simulink model "jumeau_banc_rw"  (R2025b)
settings: Solver=ode23t  StartTime=0.0  StopTime=20  MaxStep=1e-3  RelTol=1e-4
PostLoadFcn:
  | d = fileparts(get_param('jumeau_banc_rw', 'FileName')); addpath(fullfile(d, 'geometrie'), fullfile(d, 'liaison'), fullfile(d, 'pilotage')); clear d
StartFcn:
  | % Jumeau Webots : au lancement, MATLAB envoie les paramètres du Model Workspace à Webots, qui remet le banc en
  | % position de départ, puis ouvre la liaison de télémétrie et la liaison de commande (liaison/pont_banc.m).
  | if strcmp(get_param('jumeau_banc_rw/Procédé', 'LabelModeActiveChoice'), 'Webots')
  |     pont_banc('ouvrir', getVariable(get_param('jumeau_banc_rw', 'ModelWorkspace'), 'config_jumeau'));
  | end
  | pilotage_banc('depart');   % interface de pilotage : nouveau lancement
StopFcn:
  | pont_banc('fermer');
  | pilotage_banc('fin');
model workspace (MATLAB code in the model file):
  | %% Jumeau numérique du banc de stabilisation à 4 roues de réaction (version 3) : paramètres
  | % Ce code est enregistré dans le modèle (Model Explorer > jumeau_banc_rw > Model Workspace).
  | % Origine : (CAO) CAO du banc version 3, (M) mesuré sur le matériel, (F) fiche technique, (Fw) firmware,
  | % (H) hypothèse à mesurer sur le banc. Masses et inerties des pièces : dans chaque bloc de pièce.
  | 
  | %% Montage de l'essai
  | pivot_mm = 25;              % position du pivot de tangage sur le corps : 25, 24, 16, 8, 0, -8 mm (25 : banc équilibré, rangée +24 et paliers remontés de 1 mm)
  | blocage_roulis = 0;         % goupille de blocage : 1 = axe bloqué à 0°, 0 = axe libre
  | blocage_tangage = 0;
  | angle0_roulis_deg = 2;      % position de départ (mise à 0 si l'axe est bloqué)
  | angle0_tangage_deg = -1;
  | g = 9.81;                   % m/s²
  | 
  | %% Pupitre : pilotage manuel des 4 ESC
  | essai_t = 1;                % s, instant de l'échelon d'essai ajouté aux curseurs
  | essai_echelon_us = [0 0 0 0];   % µs, échelon d'essai sur chaque ESC (0 : aucun)
  | 
  | %% Alimentation des ESC
  | V_alim = 12;                % V, alimentation de labo (H : tension réglée)
  | 
  | %% ESC Brushless 30A bidirectionnels (x4)
  | f_trame_esc = 50;           % Hz, une impulsion toutes les 20 ms (Fw : LEDC 50 Hz)
  | imp_neutre = 1500;          % µs, neutre (testé sur le banc)
  | imp_min = 1000;             % µs (Fw)
  | imp_max = 2000;             % µs (Fw)
  | zone_morte_us = 0;          % µs autour du neutre (H)
  | tau_esc = 2e-3;             % s, temps de réponse de l'ESC (H)
  | armement_actif = 1;         % 1 : l'ESC ne pilote le moteur qu'après t_armement au neutre
  | t_armement = 1;             % s (H)
  | fenetre_armement_us = 25;   % µs, écart au neutre accepté pendant l'armement (H)
  | sens_moteurs = [1 1 1 1];   % +1 : au-dessus du neutre, la roue tourne dans le sens +axe (vers l'extérieur) (H : ordre des phases)
  | 
  | %% Moteurs A2212 1400 KV (x4), modèle équivalent continu
  | KV = 1400;                  % tr/min/V (F)
  | Ke = 60/(2*pi*KV);          % V.s/rad
  | Kt = Ke;                    % N.m/A
  | R_moteur = 0.08;            % ohm (H)
  | L_moteur = 30e-6;           % H (H)
  | f_roue = 5e-6;              % N.m.s/rad, frottement visqueux des roulements du moteur (H)
  | 
  | %% Cardan
  | butee_deg = 20;             % débattement de chaque axe (CAO)
  | k_butee = 20;               % N.m/rad, contact goupille-lumière (H)
  | c_butee = 0.2;              % N.m.s/rad (H)
  | b_cardan = 1e-4;            % N.m.s/rad, frottement des roulements 625 (H)
  | k_cables = 0;               % N.m/rad, raideur des deux câbles vers la table (H)
  | 
  | %% BNO055 (mode fusion)
  | T_bno = 0.01;               % s, données de fusion à 100 Hz (F)
  | bruit_bno = 1;              % 1 : bruit de mesure, 0 : capteur parfait
  | sigma_angle_deg = 0.05;     % ° (H)
  | sigma_gyro_dps = 0.1;       % °/s (H)
  | sigma_acc = 0.02;           % m/s² (H)
  | R_montage_bno = eye(3);     % axes du capteur dans le repère du dispositif : eye(3) = remappage AXIS_MAP réglé
  |                             % (la carte est tournée de 90° dans la CAO)
  | 
  | %% Capteurs de vitesse TCRT5000 (x4) : un front à chaque rayon du disque
  | n_rayons = 4;               % rayons du disque vus par tour (CAO : disque d'origine)
  | T_tcrt = 1e-3;              % s, pas de calcul du capteur (les fronts sont datés par interpolation, comme un chronomètre en µs)
  | t_arret_tcrt = 0.2;         % s sans front : la vitesse mesurée retombe à 0 (Fw, à fixer)
  | 
  | %% Pont vers le jumeau Webots (et, plus tard, vers l'ESP32 du banc réel)
  | T_pont = 0.01;              % s, une trame de commande et une trame de télémétrie toutes les 10 ms
  | 
  | %% Essai : maintien au départ et perturbation
  | t_lacher = 2;                % s, le dispositif est tenu à la main à sa position de départ jusqu'à cet instant (0 : libre dès le départ)
  | k_main = 5;                  % N.m/rad, raideur de la main qui tient le dispositif
  | c_main = 0.3;                % N.m.s/rad, son amortissement
  | perturbation_t = 7;          % s, instant de la poussée d'essai
  | perturbation_duree = 0.2;    % s
  | perturbation_couple = [0.02 0.02];   % N.m, couple de la poussée sur [roulis tangage], programmée (0 : aucune ; l'interface de pilotage en ajoute)
  | 
  | %% Grandeurs dérivées
  | assert(any(pivot_mm == [25 24 16 8 0 -8]), 'pivot_mm : 25, 24, 16, 8, 0, -8');
  | q0_deg = [angle0_roulis_deg angle0_tangage_deg] .* ([blocage_roulis blocage_tangage] == 0);
  | config_jumeau = [pivot_mm; blocage_roulis; blocage_tangage; q0_deg(:); V_alim; f_trame_esc; imp_neutre; imp_min; imp_max; ...
  |     zone_morte_us; tau_esc; armement_actif; t_armement; fenetre_armement_us; sens_moteurs(:); Ke; Kt; R_moteur; L_moteur; ...
  |     f_roue; butee_deg; k_butee; c_butee; b_cardan; k_cables; g; T_bno; bruit_bno; sigma_angle_deg; sigma_gyro_dps; ...
  |     sigma_acc; n_rayons; t_arret_tcrt; T_tcrt; R_montage_bno(:); T_pont; t_lacher; k_main; c_main];   % 51 valeurs envoyées au jumeau Webots au lancement
  | 
  | %% Commande bas niveau : une boucle de vitesse par roue, avec observateur CFO (méthode du TP2, ramenée à la vitesse)
  | J_roue = 1.562e-4;          % kg.m², inertie d'une roue autour de son axe : disque, vis, cloche du moteur (CAO)
  | T_cbn = 1/f_trame_esc;      % s, période de calcul de la commande : celle des ESC, qui ne lisent qu'une impulsion toutes les 20 ms
  | wc_roue = [10 10 10 10];    % rad/s, rapidité du suivi de vitesse de chaque roue (pôle de l'erreur en -wc)
  | wo_roue = [5 5 5 5];        % rad/s, rapidité du CFO de chaque roue (pôles en -wo et -4 wo) ; au-delà de 10, il devient instable à 20 ms
  | imp_cmd_min = 1375;         % µs, limites des impulsions commandées : vitesse conseillée des disques, 3 900 tr/min
  | imp_cmd_max = 1625;         % µs
  | w_aveugle = 45;             % rad/s, en dessous (vitesse du modèle), le TCRT5000 voit mal la roue : le CFO ne se corrige plus sur la mesure
  | 
  | %% Consigne d'essai des roues : ajoutée à la consigne qui vient de la conversion (0 tant qu'elle est vide)
  | essai_roue_t1 = 2;                  % s, départ vers le premier palier
  | essai_roue_vitesse1 = [0 0 0 0];  % rad/s, premier palier de chaque roue (0 : la roue reste à l'arrêt)
  | essai_roue_t2 = 6;                  % s, départ vers le second palier
  | essai_roue_vitesse2 = [0 0 0 0];    % rad/s, second palier de chaque roue
  | essai_roue_acc = 300;               % rad/s², pente des rampes entre les paliers
  | 
  | %% Commande bas niveau : grandeurs calculées
  | % modèle local d'une roue : d(omega)/dt = -a1 omega + a0 V + d
  | a0_roue = Kt/(R_moteur*J_roue) * [1 1 1 1];                % rad/s² par volt
  | a1_roue = (Kt*Ke/R_moteur + f_roue)/J_roue * [1 1 1 1];    % 1/s
  | K_roue = wc_roue - a1_roue;                                % retour d'état : erreur en -(a1 + K) = -wc
  | l1_roue = 5*wo_roue;                                       % CFO
  | lambda_roue = 4/5*wo_roue;
  | 
  | %% Référence : angles demandés au dispositif, en polynômes de degré 5 entre deux paliers
  | ref_t = [2 12];              % s, instant de départ vers chaque palier
  | ref_roulis_deg = [0 5];      % °, roulis demandé à chaque palier
  | ref_tangage_deg = [0 0];     % °, tangage demandé à chaque palier
  | ref_duree = 1.5;             % s, durée du passage d'un palier au suivant
  | 
  | %% Commande haut niveau : une boucle par axe [roulis tangage], placement de pôles basé sur l'observateur CFO (TP2)
  | T_chn = T_cbn;               % s, période de calcul : celle de la commande bas niveau et des ESC
  | t_depart = t_lacher;         % s, mise en marche de la commande : au moment où la main lâche le dispositif
  | wc_axe = [4 4];              % rad/s, rapidité du suivi d'angle de chaque axe
  | xi_axe = [1 1];              % amortissement
  | wo_axe = [3 3];              % rad/s, rapidité du CFO de chaque axe (pôles en -wo et -4 wo, double) ; au-delà de 4, le couple s'agite
  | desat_active = 0;            % 1 : la référence est décalée pour ramener les roues vers leur vitesse de repos
  | T_desat = 5;                 % s, constante de temps de ce retour
  | desat_max_deg = 15;          % °, décalage maximal de la référence
  | 
  | %% Conversion : couples des deux axes vers les 4 roues
  | w_repos = 200;               % rad/s, vitesse de repos des 4 roues : elles tournent toujours, le TCRT5000 les voit toujours
  | t_roues = t_armement + 0.2;  % s, mise en rotation des roues, une fois les ESC armés
  | acc_roue_max = 300;          % rad/s², accélération maximale demandée à une roue
  | w_roue_min = 60;             % rad/s, vitesses limites demandées à une roue
  | w_roue_max = 400;            % rad/s (disques : 3 900 tr/min conseillés, soit 408 rad/s)
  | 
  | %% Masses et inerties utilisées par la commande (CAO du banc version 3)
  | m_disp = 1.2615;             % kg, dispositif et ses 4 roues
  | zG_disp = 24.977e-3;         % m, hauteur de son centre de masse sur le corps (le pivot est à pivot_mm)
  | Ixx_disp_24 = 8.2684e-3;     % kg.m², inertie du dispositif autour du roulis, pivot à +24 mm
  | Iyy_disp_24 = 8.2786e-3;     % kg.m², autour du tangage, pivot à +24 mm
  | m_croix = 0.0755;            % kg, croisillon et paliers (ne tournent qu'en roulis)
  | zG_croix = 0.257e-3;         % m, hauteur de leur centre de masse au-dessus de l'axe de roulis
  | Ixx_croix = 2.073e-4;        % kg.m²
  | 
  | %% Commande haut niveau et conversion : grandeurs calculées
  | % modèle local d'un axe : d²(theta)/dt² = -a1 d(theta)/dt + a0 C + d, avec C le couple demandé aux roues
  | hz = zG_disp - pivot_mm/1000;                                    % m, centre de masse du dispositif au-dessus du pivot
  | I_axe = [Ixx_disp_24 + Ixx_croix, Iyy_disp_24] + m_disp*(hz^2 - (zG_disp - 0.024)^2) - 2*J_roue;   % kg.m²
  | mgh_axe = g*[m_disp*hz + m_croix*zG_croix, m_disp*hz];           % N.m/rad, couple de pesanteur par radian d'inclinaison
  | a0_axe = 1./I_axe;                                               % rad/s² par N.m
  | a1_axe = b_cardan./I_axe;                                        % 1/s
  | k1_axe = wc_axe.^2;                                              % retour d'état : s² + 2 xi wc s + wc²
  | k2_axe = 2*xi_axe.*wc_axe - a1_axe;
  | l1_axe = 9*wo_axe;                                               % CFO du TP2
  | l2_axe = 12*wo_axe.^2;
  | lambda_axe = 4/3*wo_axe;
  | C_max = 2*J_roue*cosd(45)*acc_roue_max;                          % N.m, couple maximal demandé sur un axe
  | k_desat = desat_active.*sign(mgh_axe + (mgh_axe == 0))./(max(abs(mgh_axe), 1e-3)*T_desat);            % rad par N.m.s
  | sx_roues = [1 -1 -1 1];                                          % signe de cos(45°, 135°, 225°, 315°) : part de chaque roue sur le roulis
  | sy_roues = [1 1 -1 -1];                                          % signe de sin : part sur le tangage
  | M_conv = -[sx_roues(:) sy_roues(:)]/(4*J_roue*cosd(45));         % accélération des 4 roues pour un couple [roulis; tangage]
  | 
  | %% Perception : des mesures à l'état du banc
  | T_perception = T_bno;        % s, période de calcul : celle du BNO055
  | tau_desequilibre = 2;        % s, constante de temps du filtre du couple extérieur et du déséquilibre
  | 
  | %% Pilotage par l'interface (pilotage/pilote_banc.m)
  | manche_max_deg = 15;         % °, limite de sécurité de l'inclinaison demandée par le manche (l'interface règle l'amplitude)
  | w_manche = 3;                % rad/s, rapidité avec laquelle la référence rejoint le manche (second ordre critique)
  | T_affichage = 0.1;           % s, rafraîchissement de l'interface
undefined symbols (not defined in the file): DiscIntNeverNeededParam, X, Y, Z
libraries: sm_lib x256, nesl_utility x24, simulink x7
(part 6 of 8)

== system jumeau_banc_rw/Procédé/Jumeau Simscape/Mécanique (CAO version 3)/Module de roue 4 (315°) ==
  A2212 stator 4 : sm_lib/Body Elements/File Solid  Description=|  ExtGeomFileName=A2212_stator.stl  UnitType=Custom  ExtGeomFileUnits=mm  StepReaderType=HEX  ExportConvexHullGeometry=off  InertiaType=Custom  BasedOnType=DensityFromFile  Density=1000  DensityUnits=kg/m^3  Mass=0.041172129  MassUnits=kg  CenterOfMass=[-3.2163675e-07 -1.5433729e-08 0.010081914]  CenterOfMassUnits=m  MomentsOfInertia=[2.9597205e-06 2.959724e-06 2.7785288e-06]  MomentsOfInertiaUnits=kg*m^2  ProductsOfInertia=[-4.4260985e-12 -1.0273354e-10 7.5029895e-09]  ProductsOfInertiaUnits=kg*m^2  GraphicType=FromGeometry  MarkerShape=Sphere  MarkerSize=10  GraphicVisPropType=SimpleVisualProperties  GraphicDiffuseColor=[0.333 0.333 0.333]  GraphicOpacity=1  GraphicSpecularColor=[0.5 0.5 0.5 1.0]  GraphicAmbientColor=[0.15 0.15 0.15 1.0]  GraphicEmissiveColor=[0.0 0.0 0.0 1.0]  GraphicShininess=75  DoExposeReferenceFrame=on  SerializedFrames=<Frames/>
      | Pièce CAO : A2212 stator 4 (A2212_stator)
      | Masse 41.17 g : tôles 7650 kg/m³, bobines cuivre, base et croix aluminium, roulements et vis acier, × 1.314 pour que le moteur pèse 58 g (fiche) : fils et connectique.
      | Centre de masse et inertie : calculés sur la géométrie de la CAO.
  Axe du moteur 4 : sm_lib/Frames and Transforms/Rigid Transform  Description=Axe Z de l'articulation = axe de l'A2212, horizontal, sur la diagonale à 315° (du centre vers l'extérieur).  RotationMethod=RotationMatrix  FollAlignAxisA=+X  BaseAlignAxisA=+Y  FollAlignAxisB=+Y  BaseAlignAxisB=+Z  RotationStandardAxis=+Z  RotationAngle=0  RotationAngleUnits=deg  RotationArbitraryAxis=[0 0 1]  RotationSequenceAxes=FollowerAxes  RotationSequence=XYX  RotationSequenceAngles=[0 0 0]  RotationSequenceAnglesUnits=deg  RotationMatrix=[0 0.707106781187 0.707106781187;0 0.707106781187 -0.707106781187;-1 0 0]  Quaternion=[1 0 0 0]  TranslationMethod=None  TranslationCartesianOffset=[0 0 0]  TranslationCartesianOffsetUnits=m  TranslationStandardAxis=+Z  TranslationStandardOffset=0  TranslationStandardOffsetUnits=m  TranslationROffset=0  TranslationROffsetUnits=m  TranslationThetaOffset=0  TranslationThetaOffsetUnits=deg  TranslationZOffset=0  TranslationZOffsetUnits=m
  Carte TCRT5000 4 : sm_lib/Body Elements/File Solid  Description=|  ExtGeomFileName=RW-33_TCRT5000.stl  UnitType=Custom  ExtGeomFileUnits=mm  StepReaderType=HEX  ExportConvexHullGeometry=off  InertiaType=Custom  BasedOnType=DensityFromFile  Density=1000  DensityUnits=kg/m^3  Mass=0.003  MassUnits=kg  CenterOfMass=[0.0016915786 -4.5510696e-20 0.00083266821]  CenterOfMassUnits=m  MomentsOfInertia=[4.9146471e-08 3.58579e-07 3.7619567e-07]  MomentsOfInertiaUnits=kg*m^2  ProductsOfInertia=[7.8340645e-25 -2.5874665e-08 6.6993709e-24]  ProductsOfInertiaUnits=kg*m^2  GraphicType=FromGeometry  MarkerShape=Sphere  MarkerSize=10  GraphicVisPropType=SimpleVisualProperties  GraphicDiffuseColor=[0.122 0.431 0.263]  GraphicOpacity=1  GraphicSpecularColor=[0.5 0.5 0.5 1.0]  GraphicAmbientColor=[0.15 0.15 0.15 1.0]  GraphicEmissiveColor=[0.0 0.0 0.0 1.0]  GraphicShininess=75  DoExposeReferenceFrame=on  SerializedFrames=<Frames/>
      | Pièce CAO : Carte TCRT5000 4 (RW-33_TCRT5000)
      | Masse 3.00 g : carte TCRT5000, estimée, 3 g répartis sur le volume de la CAO.
      | Centre de masse et inertie : calculés sur la géométrie de la CAO.
  Carter 4 : sm_lib/Body Elements/File Solid  Description=|  ExtGeomFileName=RW-03_Carter.stl  UnitType=Custom  ExtGeomFileUnits=mm  StepReaderType=HEX  ExportConvexHullGeometry=off  InertiaType=Custom  BasedOnType=DensityFromFile  Density=1000  DensityUnits=kg/m^3  Mass=0.026086558  MassUnits=kg  CenterOfMass=[-7.1999544e-18 0.0031989129 0.035794534]  CenterOfMassUnits=m  MomentsOfInertia=[6.9482784e-05 4.9569269e-05 0.00011405383]  MomentsOfInertiaUnits=kg*m^2  ProductsOfInertia=[-3.694917e-07 4.4435921e-21 1.6882936e-20]  ProductsOfInertiaUnits=kg*m^2  GraphicType=FromGeometry  MarkerShape=Sphere  MarkerSize=10  GraphicVisPropType=SimpleVisualProperties  GraphicDiffuseColor=[0.733 0.733 0.733]  GraphicOpacity=1  GraphicSpecularColor=[0.5 0.5 0.5 1.0]  GraphicAmbientColor=[0.15 0.15 0.15 1.0]  GraphicEmissiveColor=[0.0 0.0 0.0 1.0]  GraphicShininess=75  DoExposeReferenceFrame=on  SerializedFrames=<Frames/>
      | Pièce CAO : Carter 4 (RW-03_Carter)
      | Masse 26.09 g : PLA imprimé, 2 parois et 15 % de remplissage (hypothèse de conception), 800 kg/m³.
      | Centre de masse et inertie : calculés sur la géométrie de la CAO.
  Platine 4 : sm_lib/Body Elements/File Solid  Description=|  ExtGeomFileName=RW-02_Platine-moteur.stl  UnitType=Custom  ExtGeomFileUnits=mm  StepReaderType=HEX  ExportConvexHullGeometry=off  InertiaType=Custom  BasedOnType=DensityFromFile  Density=1000  DensityUnits=kg/m^3  Mass=0.011360503  MassUnits=kg  CenterOfMass=[0.0023006023 0.0040112308 0.002]  CenterOfMassUnits=m  MomentsOfInertia=[1.2693702e-05 1.288044e-06 1.3951451e-05]  MomentsOfInertiaUnits=kg*m^2  ProductsOfInertia=[-2.3283064e-23 -5.8207661e-24 -8.8833047e-07]  ProductsOfInertiaUnits=kg*m^2  GraphicType=FromGeometry  MarkerShape=Sphere  MarkerSize=10  GraphicVisPropType=SimpleVisualProperties  GraphicDiffuseColor=[0.867 0.518 0.322]  GraphicOpacity=1  GraphicSpecularColor=[0.5 0.5 0.5 1.0]  GraphicAmbientColor=[0.15 0.15 0.15 1.0]  GraphicEmissiveColor=[0.0 0.0 0.0 1.0]  GraphicShininess=75  DoExposeReferenceFrame=on  SerializedFrames=<Frames/>
      | Pièce CAO : Platine 4 (RW-02_Platine-moteur)
      | Masse 11.36 g : PLA imprimé, 2 parois et 15 % de remplissage (hypothèse de conception), 800 kg/m³.
      | Centre de masse et inertie : calculés sur la géométrie de la CAO.
  Pose A2212 stator 4 : sm_lib/Frames and Transforms/Rigid Transform  RotationMethod=RotationMatrix  FollAlignAxisA=+X  BaseAlignAxisA=+Y  FollAlignAxisB=+Y  BaseAlignAxisB=+Z  RotationStandardAxis=+Z  RotationAngle=0  RotationAngleUnits=deg  RotationArbitraryAxis=[0 0 1]  RotationSequenceAxes=FollowerAxes  RotationSequence=XYX  RotationSequenceAngles=[0 0 0]  RotationSequenceAnglesUnits=deg  RotationMatrix=[0.7071067812 0 0.7071067812;0.7071067812 0 -0.7071067812;0 1 0]  Quaternion=[1 0 0 0]  TranslationMethod=Cartesian  TranslationCartesianOffset=[60.811183 -60.811183 0]  TranslationCartesianOffsetUnits=mm  TranslationStandardAxis=+Z  TranslationStandardOffset=0  TranslationStandardOffsetUnits=m  TranslationROffset=0  TranslationROffsetUnits=m  TranslationThetaOffset=0  TranslationThetaOffsetUnits=deg  TranslationZOffset=0  TranslationZOffsetUnits=m
  Pose Carte TCRT5000 4 : sm_lib/Frames and Transforms/Rigid Transform  RotationMethod=RotationMatrix  FollAlignAxisA=+X  BaseAlignAxisA=+Y  FollAlignAxisB=+Y  BaseAlignAxisB=+Z  RotationStandardAxis=+Z  RotationAngle=0  RotationAngleUnits=deg  RotationArbitraryAxis=[0 0 1]  RotationSequenceAxes=FollowerAxes  RotationSequence=XYX  RotationSequenceAngles=[0 0 0]  RotationSequenceAnglesUnits=deg  RotationMatrix=[0.7071067812 0 -0.7071067812;0.7071067812 0 0.7071067812;0 -1 0]  Quaternion=[1 0 0 0]  TranslationMethod=Cartesian  TranslationCartesianOffset=[93.479516 -93.479516 40]  TranslationCartesianOffsetUnits=mm  TranslationStandardAxis=+Z  TranslationStandardOffset=0  TranslationStandardOffsetUnits=m  TranslationROffset=0  TranslationROffsetUnits=m  TranslationThetaOffset=0  TranslationThetaOffsetUnits=deg  TranslationZOffset=0  TranslationZOffsetUnits=m
  Pose Carter 4 : sm_lib/Frames and Transforms/Rigid Transform  RotationMethod=RotationMatrix  FollAlignAxisA=+X  BaseAlignAxisA=+Y  FollAlignAxisB=+Y  BaseAlignAxisB=+Z  RotationStandardAxis=+Z  RotationAngle=0  RotationAngleUnits=deg  RotationArbitraryAxis=[0 0 1]  RotationSequenceAxes=FollowerAxes  RotationSequence=XYX  RotationSequenceAngles=[0 0 0]  RotationSequenceAnglesUnits=deg  RotationMatrix=[0.7071067812 0 0.7071067812;0.7071067812 0 -0.7071067812;0 1 0]  Quaternion=[1 0 0 0]  TranslationMethod=Cartesian  TranslationCartesianOffset=[56.568542 -56.568542 0]  TranslationCartesianOffsetUnits=mm  TranslationStandardAxis=+Z  TranslationStandardOffset=0  TranslationStandardOffsetUnits=m  TranslationROffset=0  TranslationROffsetUnits=m  TranslationThetaOffset=0  TranslationThetaOffsetUnits=deg  TranslationZOffset=0  TranslationZOffsetUnits=m
  Pose Platine 4 : sm_lib/Frames and Transforms/Rigid Transform  RotationMethod=RotationMatrix  FollAlignAxisA=+X  BaseAlignAxisA=+Y  FollAlignAxisB=+Y  BaseAlignAxisB=+Z  RotationStandardAxis=+Z  RotationAngle=0  RotationAngleUnits=deg  RotationArbitraryAxis=[0 0 1]  RotationSequenceAxes=FollowerAxes  RotationSequence=XYX  RotationSequenceAngles=[0 0 0]  RotationSequenceAnglesUnits=deg  RotationMatrix=[0.7071067812 0 0.7071067812;0.7071067812 0 -0.7071067812;0 1 0]  Quaternion=[1 0 0 0]  TranslationMethod=Cartesian  TranslationCartesianOffset=[56.568542 -56.568542 0]  TranslationCartesianOffsetUnits=mm  TranslationStandardAxis=+Z  TranslationStandardOffset=0  TranslationStandardOffsetUnits=m  TranslationROffset=0  TranslationROffsetUnits=m  TranslationThetaOffset=0  TranslationThetaOffsetUnits=deg  TranslationZOffset=0  TranslationZOffsetUnits=m
  Pose Potence 4 : sm_lib/Frames and Transforms/Rigid Transform  RotationMethod=RotationMatrix  FollAlignAxisA=+X  BaseAlignAxisA=+Y  FollAlignAxisB=+Y  BaseAlignAxisB=+Z  RotationStandardAxis=+Z  RotationAngle=0  RotationAngleUnits=deg  RotationArbitraryAxis=[0 0 1]  RotationSequenceAxes=FollowerAxes  RotationSequence=XYX  RotationSequenceAngles=[0 0 0]  RotationSequenceAnglesUnits=deg  RotationMatrix=[0.7071067812 0 0.7071067812;0.7071067812 0 -0.7071067812;0 1 0]  Quaternion=[1 0 0 0]  TranslationMethod=Cartesian  TranslationCartesianOffset=[56.568542 -56.568542 0]  TranslationCartesianOffsetUnits=mm  TranslationStandardAxis=+Z  TranslationStandardOffset=0  TranslationStandardOffsetUnits=m  TranslationROffset=0  TranslationROffsetUnits=m  TranslationThetaOffset=0  TranslationThetaOffsetUnits=deg  TranslationZOffset=0  TranslationZOffsetUnits=m
  Potence 4 : sm_lib/Body Elements/File Solid  Description=|  ExtGeomFileName=RW-12_Potence-capteur.stl  UnitType=Custom  ExtGeomFileUnits=mm  StepReaderType=HEX  ExportConvexHullGeometry=off  InertiaType=Custom  BasedOnType=DensityFromFile  Density=1000  DensityUnits=kg/m^3  Mass=0.0020458839  MassUnits=kg  CenterOfMass=[3.6184688e-20 0.062495169 0.051676295]  CenterOfMassUnits=m  MomentsOfInertia=[4.8939905e-07 1.3018391e-07 4.0974246e-07]  MomentsOfInertiaUnits=kg*m^2  ProductsOfInertia=[1.0971683e-07 -7.0286717e-24 -4.2688313e-25]  ProductsOfInertiaUnits=kg*m^2  GraphicType=FromGeometry  MarkerShape=Sphere  MarkerSize=10  GraphicVisPropType=SimpleVisualProperties  GraphicDiffuseColor=[0.91 0.639 0.239]  GraphicOpacity=1  GraphicSpecularColor=[0.5 0.5 0.5 1.0]  GraphicAmbientColor=[0.15 0.15 0.15 1.0]  GraphicEmissiveColor=[0.0 0.0 0.0 1.0]  GraphicShininess=75  DoExposeReferenceFrame=on  SerializedFrames=<Frames/>
      | Pièce CAO : Potence 4 (RW-12_Potence-capteur)
      | Masse 2.05 g : PLA imprimé, 2 parois et 15 % de remplissage (hypothèse de conception), 800 kg/m³.
      | Centre de masse et inertie : calculés sur la géométrie de la CAO.
  "Rotor 4 (disque, vis, rotor A2212)" : Subsystem  Description=repère : axe du moteur (Z), origine au centre du dispositif
  Roue 4 : sm_lib/Joints/Revolute Joint  Description=Roulements de l'A2212 : couple moteur Cm en entrée ; angle et vitesse de la roue par rapport au dispositif en sortie ; frottement f_roue.  JointMode=Normal  CompositeWrenchDir=FollowerOnBase  CompositeWrenchFrame=BaseFrame  SenseConstraintForce=off  SenseConstraintTorque=off  SenseTotalForce=off  SenseTotalTorque=off  PositionTargetSpecify=off  PositionTargetPriority=High  PositionTargetValue=0  PositionTargetValueUnits=deg  VelocityTargetSpecify=off  VelocityTargetPriority=High  VelocityTargetValue=0  VelocityTargetValueUnits=deg/s  EquilibriumPosition=0  EquilibriumPositionUnits=deg  SpringStiffness=0  SpringStiffnessUnits=N*m/deg  DampingCoefficient=f_roue  DampingCoefficientUnits=N*m*s/rad  LowerLimitSpecify=off  LowerLimitBound=-90  LowerLimitBoundUnits=deg  LowerLimitStiffness=1e4  LowerLimitStiffnessUnits=N*m/deg  LowerLimitDamping=10  LowerLimitDampingUnits=N*m/(deg/s)  LowerLimitTransitionRegionWidth=0.1  LowerLimitTransitionRegionWidthUnits=deg  UpperLimitSpecify=off  UpperLimitBound=90  UpperLimitBoundUnits=deg  UpperLimitStiffness=1e4  UpperLimitStiffnessUnits=N*m/deg  UpperLimitDamping=10  UpperLimitDampingUnits=N*m/(deg/s)  UpperLimitTransitionRegionWidth=0.1  UpperLimitTransitionRegionWidthUnits=deg  TorqueActuationMode=InputTorque  MotionActuationMode=ComputedMotion  SensePosition=on  SenseVelocity=on  SenseAcceleration=off  SenseTorqueForce=off  SenseLowerLimitTorqueForce=off  SenseUpperLimitTorqueForce=off
  D : PMIOPort  Side=Left
  Cm : PMIOPort  Port=2  Side=Left
  omega : PMIOPort  Port=3  Side=Right
  theta : PMIOPort  Port=4  Side=Right
  connections:
  Pose Platine 4/LConn1 -- D/RConn1 -- Pose Carter 4/LConn1 -- Pose Potence 4/LConn1 -- Pose Carte TCRT5000 4/LConn1 -- Pose A2212 stator 4/LConn1 -- Axe du moteur 4/LConn1
  Pose Platine 4/RConn1 -- Platine 4/RConn1
  Pose Carter 4/RConn1 -- Carter 4/RConn1
  Pose Potence 4/RConn1 -- Potence 4/RConn1
  Pose Carte TCRT5000 4/RConn1 -- Carte TCRT5000 4/RConn1
  Pose A2212 stator 4/RConn1 -- A2212 stator 4/RConn1
  Axe du moteur 4/RConn1 -- Roue 4/LConn1
  Cm/RConn1 -- Roue 4/LConn2
  Roue 4/RConn2 -- theta/RConn1
  Roue 4/RConn3 -- omega/RConn1
  Roue 4/RConn1 -- "Rotor 4 (disque, vis, rotor A2212)"/LConn1

== system jumeau_banc_rw/Procédé/Jumeau Simscape/Mécanique (CAO version 3)/Paliers de tangage ==
  Palier 1 : sm_lib/Body Elements/File Solid  Description=|  ExtGeomFileName=RW-04_Palier.stl  UnitType=Custom  ExtGeomFileUnits=mm  StepReaderType=HEX  ExportConvexHullGeometry=off  InertiaType=Custom  BasedOnType=DensityFromFile  Density=1000  DensityUnits=kg/m^3  Mass=0.0079402814  MassUnits=kg  CenterOfMass=[-3.1445323e-19 -0.00024057291 0.0038712388]  CenterOfMassUnits=m  MomentsOfInertia=[1.5342689e-06 8.8243228e-07 2.330905e-06]  MomentsOfInertiaUnits=kg*m^2  ProductsOfInertia=[2.4596172e-10 -4.9136393e-25 -2.83106e-23]  ProductsOfInertiaUnits=kg*m^2  GraphicType=FromGeometry  MarkerShape=Sphere  MarkerSize=10  GraphicVisPropType=SimpleVisualProperties  GraphicDiffuseColor=[0.867 0.518 0.322]  GraphicOpacity=1  GraphicSpecularColor=[0.5 0.5 0.5 1.0]  GraphicAmbientColor=[0.15 0.15 0.15 1.0]  GraphicEmissiveColor=[0.0 0.0 0.0 1.0]  GraphicShininess=75  DoExposeReferenceFrame=on  SerializedFrames=<Frames/>
      | Pièce CAO : Palier 1 (RW-04_Palier)
      | Masse 7.94 g : PLA imprimé, 2 parois et 15 % de remplissage (hypothèse de conception), 800 kg/m³.
      | Centre de masse et inertie : calculés sur la géométrie de la CAO.
  Palier 2 : sm_lib/Body Elements/File Solid  Description=|  ExtGeomFileName=RW-04_Palier.stl  UnitType=Custom  ExtGeomFileUnits=mm  StepReaderType=HEX  ExportConvexHullGeometry=off  InertiaType=Custom  BasedOnType=DensityFromFile  Density=1000  DensityUnits=kg/m^3  Mass=0.0079402814  MassUnits=kg  CenterOfMass=[-3.1445323e-19 -0.00024057291 0.0038712388]  CenterOfMassUnits=m  MomentsOfInertia=[1.5342689e-06 8.8243228e-07 2.330905e-06]  MomentsOfInertiaUnits=kg*m^2  ProductsOfInertia=[2.4596172e-10 -4.9136393e-25 -2.83106e-23]  ProductsOfInertiaUnits=kg*m^2  GraphicType=FromGeometry  MarkerShape=Sphere  MarkerSize=10  GraphicVisPropType=SimpleVisualProperties  GraphicDiffuseColor=[0.867 0.518 0.322]  GraphicOpacity=1  GraphicSpecularColor=[0.5 0.5 0.5 1.0]  GraphicAmbientColor=[0.15 0.15 0.15 1.0]  GraphicEmissiveColor=[0.0 0.0 0.0 1.0]  GraphicShininess=75  DoExposeReferenceFrame=on  SerializedFrames=<Frames/>
      | Pièce CAO : Palier 2 (RW-04_Palier)
      | Masse 7.94 g : PLA imprimé, 2 parois et 15 % de remplissage (hypothèse de conception), 800 kg/m³.
      | Centre de masse et inertie : calculés sur la géométrie de la CAO.
  Pose Palier 1 : sm_lib/Frames and Transforms/Rigid Transform  RotationMethod=RotationMatrix  FollAlignAxisA=+X  BaseAlignAxisA=+Y  FollAlignAxisB=+Y  BaseAlignAxisB=+Z  RotationStandardAxis=+Z  RotationAngle=0  RotationAngleUnits=deg  RotationArbitraryAxis=[0 0 1]  RotationSequenceAxes=FollowerAxes  RotationSequence=XYX  RotationSequenceAngles=[0 0 0]  RotationSequenceAnglesUnits=deg  RotationMatrix=[-1 0 0;0 0 1;0 1 0]  Quaternion=[1 0 0 0]  TranslationMethod=Cartesian  TranslationCartesianOffset=[0 80 0]  TranslationCartesianOffsetUnits=mm  TranslationStandardAxis=+Z  TranslationStandardOffset=0  TranslationStandardOffsetUnits=m  TranslationROffset=0  TranslationROffsetUnits=m  TranslationThetaOffset=0  TranslationThetaOffsetUnits=deg  TranslationZOffset=0  TranslationZOffsetUnits=m
  Pose Palier 2 : sm_lib/Frames and Transforms/Rigid Transform  RotationMethod=RotationMatrix  FollAlignAxisA=+X  BaseAlignAxisA=+Y  FollAlignAxisB=+Y  BaseAlignAxisB=+Z  RotationStandardAxis=+Z  RotationAngle=0  RotationAngleUnits=deg  RotationArbitraryAxis=[0 0 1]  RotationSequenceAxes=FollowerAxes  RotationSequence=XYX  RotationSequenceAngles=[0 0 0]  RotationSequenceAnglesUnits=deg  RotationMatrix=[1 0 0;0 0 -1;0 1 0]  Quaternion=[1 0 0 0]  TranslationMethod=Cartesian  TranslationCartesianOffset=[0 -80 0]  TranslationCartesianOffsetUnits=mm  TranslationStandardAxis=+Z  TranslationStandardOffset=0  TranslationStandardOffsetUnits=m  TranslationROffset=0  TranslationROffsetUnits=m  TranslationThetaOffset=0  TranslationThetaOffsetUnits=deg  TranslationZOffset=0  TranslationZOffsetUnits=m
  Pose Roulement de tangage 1 : sm_lib/Frames and Transforms/Rigid Transform  RotationMethod=RotationMatrix  FollAlignAxisA=+X  BaseAlignAxisA=+Y  FollAlignAxisB=+Y  BaseAlignAxisB=+Z  RotationStandardAxis=+Z  RotationAngle=0  RotationAngleUnits=deg  RotationArbitraryAxis=[0 0 1]  RotationSequenceAxes=FollowerAxes  RotationSequence=XYX  RotationSequenceAngles=[0 0 0]  RotationSequenceAnglesUnits=deg  RotationMatrix=[-1 0 0;0 0 1;0 1 0]  Quaternion=[1 0 0 0]  TranslationMethod=Cartesian  TranslationCartesianOffset=[0 83 0]  TranslationCartesianOffsetUnits=mm  TranslationStandardAxis=+Z  TranslationStandardOffset=0  TranslationStandardOffsetUnits=m  TranslationROffset=0  TranslationROffsetUnits=m  TranslationThetaOffset=0  TranslationThetaOffsetUnits=deg  TranslationZOffset=0  TranslationZOffsetUnits=m
  Pose Roulement de tangage 2 : sm_lib/Frames and Transforms/Rigid Transform  RotationMethod=RotationMatrix  FollAlignAxisA=+X  BaseAlignAxisA=+Y  FollAlignAxisB=+Y  BaseAlignAxisB=+Z  RotationStandardAxis=+Z  RotationAngle=0  RotationAngleUnits=deg  RotationArbitraryAxis=[0 0 1]  RotationSequenceAxes=FollowerAxes  RotationSequence=XYX  RotationSequenceAngles=[0 0 0]  RotationSequenceAnglesUnits=deg  RotationMatrix=[1 0 0;0 0 -1;0 1 0]  Quaternion=[1 0 0 0]  TranslationMethod=Cartesian  TranslationCartesianOffset=[0 -83 0]  TranslationCartesianOffsetUnits=mm  TranslationStandardAxis=+Z  TranslationStandardOffset=0  TranslationStandardOffsetUnits=m  TranslationROffset=0  TranslationROffsetUnits=m  TranslationThetaOffset=0  TranslationThetaOffsetUnits=deg  TranslationZOffset=0  TranslationZOffsetUnits=m
  Roulement de tangage 1 : sm_lib/Body Elements/File Solid  Description=|  ExtGeomFileName=RW-20_Roulement-625.stl  UnitType=Custom  ExtGeomFileUnits=mm  StepReaderType=HEX  ExportConvexHullGeometry=off  InertiaType=Custom  BasedOnType=DensityFromFile  Density=1000  DensityUnits=kg/m^3  Mass=0.0044  MassUnits=kg  CenterOfMass=[-4.3080529e-19 -4.0130534e-19 0.0025]  CenterOfMassUnits=m  MomentsOfInertia=[8.6441667e-08 8.6441667e-08 1.5455e-07]  MomentsOfInertiaUnits=kg*m^2  ProductsOfInertia=[-6.0797928e-26 -7.409851e-25 8.4651334e-24]  ProductsOfInertiaUnits=kg*m^2  GraphicType=FromGeometry  MarkerShape=Sphere  MarkerSize=10  GraphicVisPropType=SimpleVisualProperties  GraphicDiffuseColor=[0.627 0.627 0.627]  GraphicOpacity=1  GraphicSpecularColor=[0.5 0.5 0.5 1.0]  GraphicAmbientColor=[0.15 0.15 0.15 1.0]  GraphicEmissiveColor=[0.0 0.0 0.0 1.0]  GraphicShininess=75  DoExposeReferenceFrame=on  SerializedFrames=<Frames/>
      | Pièce CAO : Roulement de tangage 1 (RW-20_Roulement-625)
      | Masse 4.40 g : roulement 625, catalogue, 4,4 g répartis sur le volume de la CAO.
      | Centre de masse et inertie : calculés sur la géométrie de la CAO.
  Roulement de tangage 2 : sm_lib/Body Elements/File Solid  Description=|  ExtGeomFileName=RW-20_Roulement-625.stl  UnitType=Custom  ExtGeomFileUnits=mm  StepReaderType=HEX  ExportConvexHullGeometry=off  InertiaType=Custom  BasedOnType=DensityFromFile  Density=1000  DensityUnits=kg/m^3  Mass=0.0044  MassUnits=kg  CenterOfMass=[-4.3080529e-19 -4.0130534e-19 0.0025]  CenterOfMassUnits=m  MomentsOfInertia=[8.6441667e-08 8.6441667e-08 1.5455e-07]  MomentsOfInertiaUnits=kg*m^2  ProductsOfInertia=[-6.0797928e-26 -7.409851e-25 8.4651334e-24]  ProductsOfInertiaUnits=kg*m^2  GraphicType=FromGeometry  MarkerShape=Sphere  MarkerSize=10  GraphicVisPropType=SimpleVisualProperties  GraphicDiffuseColor=[0.627 0.627 0.627]  GraphicOpacity=1  GraphicSpecularColor=[0.5 0.5 0.5 1.0]  GraphicAmbientColor=[0.15 0.15 0.15 1.0]  GraphicEmissiveColor=[0.0 0.0 0.0 1.0]  GraphicShininess=75  DoExposeReferenceFrame=on  SerializedFrames=<Frames/>
      | Pièce CAO : Roulement de tangage 2 (RW-20_Roulement-625)
      | Masse 4.40 g : roulement 625, catalogue, 4,4 g répartis sur le volume de la CAO.
      | Centre de masse et inertie : calculés sur la géométrie de la CAO.
  F : PMIOPort  Side=Left
  connections:
  Pose Palier 1/LConn1 -- F/RConn1 -- Pose Roulement de tangage 1/LConn1 -- Pose Palier 2/LConn1 -- Pose Roulement de tangage 2/LConn1
  Pose Palier 1/RConn1 -- Palier 1/RConn1
  Pose Roulement de tangage 1/RConn1 -- Roulement de tangage 1/RConn1
  Pose Palier 2/RConn1 -- Palier 2/RConn1
  Pose Roulement de tangage 2/RConn1 -- Roulement de tangage 2/RConn1

== system jumeau_banc_rw/Procédé/Jumeau Simscape/Mécanique (CAO version 3)/Poussée et tenue à la main ==
  note: Couple extérieur sur le roulis et sur le tangage, pour les essais.
      | Tenue à la main : jusqu'à t_lacher, un ressort amorti (k_main, c_main) garde le dispositif à sa position de départ.
      | Poussée : couple d'essai venu du bloc « Poussée d'essai » du niveau haut (poussée programmée et poussées de l'interface de pilotage).
  angles du cardan (°) : Inport
  vitesses du cardan (° par s) : Inport  Port=2
  poussée (N.m) : Inport  Port=3
  Amortissement de la main : Gain  Gain=c_main*pi/180
  Couple de la main : Sum  Inputs=+-
  Couple extérieur : Sum
  Position de départ : Constant  Value=q0_deg(:)
  Raideur de la main : Gain  Gain=k_main*pi/180
  Tenu jusqu'à t_lacher : Step  Time=t_lacher  Before=1  After=0  SampleTime=0
  x tenu : Product
  Écart à la position de départ : Sum  Inputs=+-
  couple sur les axes (N.m) : Outport
  wires:
  Position de départ/1 -> Écart à la position de départ/1
  angles du cardan (°)/1 -> Écart à la position de départ/2
  Écart à la position de départ/1 -> Raideur de la main/1
  vitesses du cardan (° par s)/1 -> Amortissement de la main/1
  Raideur de la main/1 -> Couple de la main/1
  Amortissement de la main/1 -> Couple de la main/2
  Couple de la main/1 -> x tenu/1
  Tenu jusqu'à t_lacher/1 -> x tenu/2
  x tenu/1 -> Couple extérieur/1
  Couple extérieur/1 -> couple sur les axes (N.m)/1
  poussée (N.m)/1 -> Couple extérieur/2

== system jumeau_banc_rw/Procédé/Jumeau Simscape/Mécanique (CAO version 3)/Module de roue 1 (45°)/Rotor 1 (disque, vis, rotor A2212) ==
  A2212 rotor (roue 1) : sm_lib/Body Elements/File Solid  Description=|  ExtGeomFileName=A2212_rotor.stl  UnitType=Custom  ExtGeomFileUnits=mm  StepReaderType=HEX  ExportConvexHullGeometry=off  InertiaType=Custom  BasedOnType=DensityFromFile  Density=1000  DensityUnits=kg/m^3  Mass=0.016827871  MassUnits=kg  CenterOfMass=[2.4267094e-06 -3.2856014e-08 0.015974753]  CenterOfMassUnits=m  MomentsOfInertia=[1.7900011e-06 1.7901749e-06 1.9632852e-06]  MomentsOfInertiaUnits=kg*m^2  ProductsOfInertia=[3.6666561e-12 -1.1397813e-09 -5.9134076e-14]  ProductsOfInertiaUnits=kg*m^2  GraphicType=FromGeometry  MarkerShape=Sphere  MarkerSize=10  GraphicVisPropType=SimpleVisualProperties  GraphicDiffuseColor=[0.549 0.549 0.549]  GraphicOpacity=1  GraphicSpecularColor=[0.5 0.5 0.5 1.0]  GraphicAmbientColor=[0.15 0.15 0.15 1.0]  GraphicEmissiveColor=[0.0 0.0 0.0 1.0]  GraphicShininess=75  DoExposeReferenceFrame=on  SerializedFrames=<Frames/>
      | Pièce CAO : A2212 rotor (roue 1) (A2212_rotor)
      | Masse 16.83 g : cloche aluminium, 14 aimants NdFeB 7500 kg/m³, arbre, vis pointeau et circlip acier.
      | Centre de masse et inertie : calculés sur la géométrie de la CAO.
  Pose A2212 rotor (roue 1) : sm_lib/Frames and Transforms/Rigid Transform  RotationMethod=RotationMatrix  FollAlignAxisA=+X  BaseAlignAxisA=+Y  FollAlignAxisB=+Y  BaseAlignAxisB=+Z  RotationStandardAxis=+Z  RotationAngle=0  RotationAngleUnits=deg  RotationArbitraryAxis=[0 0 1]  RotationSequenceAxes=FollowerAxes  RotationSequence=XYX  RotationSequenceAngles=[0 0 0]  RotationSequenceAnglesUnits=deg  RotationMatrix=[0 -1 0;1 0 0;0 0 1]  Quaternion=[1 0 0 0]  TranslationMethod=Cartesian  TranslationCartesianOffset=[0 0.001192 86]  TranslationCartesianOffsetUnits=mm  TranslationStandardAxis=+Z  TranslationStandardOffset=0  TranslationStandardOffsetUnits=m  TranslationROffset=0  TranslationROffsetUnits=m  TranslationThetaOffset=0  TranslationThetaOffsetUnits=deg  TranslationZOffset=0  TranslationZOffsetUnits=m
  Pose disque-1 (roue 1) : sm_lib/Frames and Transforms/Rigid Transform  RotationMethod=RotationMatrix  FollAlignAxisA=+X  BaseAlignAxisA=+Y  FollAlignAxisB=+Y  BaseAlignAxisB=+Z  RotationStandardAxis=+Z  RotationAngle=0  RotationAngleUnits=deg  RotationArbitraryAxis=[0 0 1]  RotationSequenceAxes=FollowerAxes  RotationSequence=XYX  RotationSequenceAngles=[0 0 0]  RotationSequenceAnglesUnits=deg  RotationMatrix=[0 -1 0;1 0 0;0 0 1]  Quaternion=[1 0 0 0]  TranslationMethod=Cartesian  TranslationCartesianOffset=[0 0 116.7]  TranslationCartesianOffsetUnits=mm  TranslationStandardAxis=+Z  TranslationStandardOffset=0  TranslationStandardOffsetUnits=m  TranslationROffset=0  TranslationROffsetUnits=m  TranslationThetaOffset=0  TranslationThetaOffsetUnits=deg  TranslationZOffset=0  TranslationZOffsetUnits=m
  Pose ecrous-1 (roue 1) : sm_lib/Frames and Transforms/Rigid Transform  RotationMethod=RotationMatrix  FollAlignAxisA=+X  BaseAlignAxisA=+Y  FollAlignAxisB=+Y  BaseAlignAxisB=+Z  RotationStandardAxis=+Z  RotationAngle=0  RotationAngleUnits=deg  RotationArbitraryAxis=[0 0 1]  RotationSequenceAxes=FollowerAxes  RotationSequence=XYX  RotationSequenceAngles=[0 0 0]  RotationSequenceAnglesUnits=deg  RotationMatrix=[0 -1 0;1 0 0;0 0 1]  Quaternion=[1 0 0 0]  TranslationMethod=Cartesian  TranslationCartesianOffset=[0 -55 110.7]  TranslationCartesianOffsetUnits=mm  TranslationStandardAxis=+Z  TranslationStandardOffset=0  TranslationStandardOffsetUnits=m  TranslationROffset=0  TranslationROffsetUnits=m  TranslationThetaOffset=0  TranslationThetaOffsetUnits=deg  TranslationZOffset=0  TranslationZOffsetUnits=m
  Pose ecrous-2 (roue 1) : sm_lib/Frames and Transforms/Rigid Transform  RotationMethod=RotationMatrix  FollAlignAxisA=+X  BaseAlignAxisA=+Y  FollAlignAxisB=+Y  BaseAlignAxisB=+Z  RotationStandardAxis=+Z  RotationAngle=0  RotationAngleUnits=deg  RotationArbitraryAxis=[0 0 1]  RotationSequenceAxes=FollowerAxes  RotationSequence=XYX  RotationSequenceAngles=[0 0 0]  RotationSequenceAnglesUnits=deg  RotationMatrix=[0 -1 0;1 0 0;0 0 1]  Quaternion=[1 0 0 0]  TranslationMethod=Cartesian  TranslationCartesianOffset=[55 0 110.7]  TranslationCartesianOffsetUnits=mm  TranslationStandardAxis=+Z  TranslationStandardOffset=0  TranslationStandardOffsetUnits=m  TranslationROffset=0  TranslationROffsetUnits=m  TranslationThetaOffset=0  TranslationThetaOffsetUnits=deg  TranslationZOffset=0  TranslationZOffsetUnits=m
  Pose ecrous-3 (roue 1) : sm_lib/Frames and Transforms/Rigid Transform  RotationMethod=RotationMatrix  FollAlignAxisA=+X  BaseAlignAxisA=+Y  FollAlignAxisB=+Y  BaseAlignAxisB=+Z  RotationStandardAxis=+Z  RotationAngle=0  RotationAngleUnits=deg  RotationArbitraryAxis=[0 0 1]  RotationSequenceAxes=FollowerAxes  RotationSequence=XYX  RotationSequenceAngles=[0 0 0]  RotationSequenceAnglesUnits=deg  RotationMatrix=[0 -1 0;1 0 0;0 0 1]  Quaternion=[1 0 0 0]  TranslationMethod=Cartesian  TranslationCartesianOffset=[-55 0 110.7]  TranslationCartesianOffsetUnits=mm  TranslationStandardAxis=+Z  TranslationStandardOffset=0  TranslationStandardOffsetUnits=m  TranslationROffset=0  TranslationROffsetUnits=m  TranslationThetaOffset=0  TranslationThetaOffsetUnits=deg  TranslationZOffset=0  TranslationZOffsetUnits=m
  Pose ecrous-4 (roue 1) : sm_lib/Frames and Transforms/Rigid Transform  RotationMethod=RotationMatrix  FollAlignAxisA=+X  BaseAlignAxisA=+Y  FollAlignAxisB=+Y  BaseAlignAxisB=+Z  RotationStandardAxis=+Z  RotationAngle=0  RotationAngleUnits=deg  RotationArbitraryAxis=[0 0 1]  RotationSequenceAxes=FollowerAxes  RotationSequence=XYX  RotationSequenceAngles=[0 0 0]  RotationSequenceAnglesUnits=deg  RotationMatrix=[0 -1 0;1 0 0;0 0 1]  Quaternion=[1 0 0 0]  TranslationMethod=Cartesian  TranslationCartesianOffset=[0 55 110.7]  TranslationCartesianOffsetUnits=mm  TranslationStandardAxis=+Z  TranslationStandardOffset=0  TranslationStandardOffsetUnits=m  TranslationROffset=0  TranslationROffsetUnits=m  TranslationThetaOffset=0  TranslationThetaOffsetUnits=deg  TranslationZOffset=0  TranslationZOffsetUnits=m
  Pose vis10-1 (roue 1) : sm_lib/Frames and Transforms/Rigid Transform  RotationMethod=RotationMatrix  FollAlignAxisA=+X  BaseAlignAxisA=+Y  FollAlignAxisB=+Y  BaseAlignAxisB=+Z  RotationStandardAxis=+Z  RotationAngle=0  RotationAngleUnits=deg  RotationArbitraryAxis=[0 0 1]  RotationSequenceAxes=FollowerAxes  RotationSequence=XYX  RotationSequenceAngles=[0 0 0]  RotationSequenceAnglesUnits=deg  RotationMatrix=[0 -1 0;1 0 0;0 0 1]  Quaternion=[1 0 0 0]  TranslationMethod=Cartesian  TranslationCartesianOffset=[55 0 111.2]  TranslationCartesianOffsetUnits=mm  TranslationStandardAxis=+Z  TranslationStandardOffset=0  TranslationStandardOffsetUnits=m  TranslationROffset=0  TranslationROffsetUnits=m  TranslationThetaOffset=0  TranslationThetaOffsetUnits=deg  TranslationZOffset=0  TranslationZOffsetUnits=m
  Pose vis10-2 (roue 1) : sm_lib/Frames and Transforms/Rigid Transform  RotationMethod=RotationMatrix  FollAlignAxisA=+X  BaseAlignAxisA=+Y  FollAlignAxisB=+Y  BaseAlignAxisB=+Z  RotationStandardAxis=+Z  RotationAngle=0  RotationAngleUnits=deg  RotationArbitraryAxis=[0 0 1]  RotationSequenceAxes=FollowerAxes  RotationSequence=XYX  RotationSequenceAngles=[0 0 0]  RotationSequenceAnglesUnits=deg  RotationMatrix=[0 -1 0;1 0 0;0 0 1]  Quaternion=[1 0 0 0]  TranslationMethod=Cartesian  TranslationCartesianOffset=[-55 0 111.2]  TranslationCartesianOffsetUnits=mm  TranslationStandardAxis=+Z  TranslationStandardOffset=0  TranslationStandardOffsetUnits=m  TranslationROffset=0  TranslationROffsetUnits=m  TranslationThetaOffset=0  TranslationThetaOffsetUnits=deg  TranslationZOffset=0  TranslationZOffsetUnits=m
  Pose vis20-1 (roue 1) : sm_lib/Frames and Transforms/Rigid Transform  RotationMethod=RotationMatrix  FollAlignAxisA=+X  BaseAlignAxisA=+Y  FollAlignAxisB=+Y  BaseAlignAxisB=+Z  RotationStandardAxis=+Z  RotationAngle=0  RotationAngleUnits=deg  RotationArbitraryAxis=[0 0 1]  RotationSequenceAxes=FollowerAxes  RotationSequence=XYX  RotationSequenceAngles=[0 0 0]  RotationSequenceAnglesUnits=deg  RotationMatrix=[0 -1 0;1 0 0;0 0 1]  Quaternion=[1 0 0 0]  TranslationMethod=Cartesian  TranslationCartesianOffset=[0 55 101.2]  TranslationCartesianOffsetUnits=mm  TranslationStandardAxis=+Z  TranslationStandardOffset=0  TranslationStandardOffsetUnits=m  TranslationROffset=0  TranslationROffsetUnits=m  TranslationThetaOffset=0  TranslationThetaOffsetUnits=deg  TranslationZOffset=0  TranslationZOffsetUnits=m
  Pose vis20-2 (roue 1) : sm_lib/Frames and Transforms/Rigid Transform  RotationMethod=RotationMatrix  FollAlignAxisA=+X  BaseAlignAxisA=+Y  FollAlignAxisB=+Y  BaseAlignAxisB=+Z  RotationStandardAxis=+Z  RotationAngle=0  RotationAngleUnits=deg  RotationArbitraryAxis=[0 0 1]  RotationSequenceAxes=FollowerAxes  RotationSequence=XYX  RotationSequenceAngles=[0 0 0]  RotationSequenceAnglesUnits=deg  RotationMatrix=[0 -1 0;1 0 0;0 0 1]  Quaternion=[1 0 0 0]  TranslationMethod=Cartesian  TranslationCartesianOffset=[0 -55 99.853166]  TranslationCartesianOffsetUnits=mm  TranslationStandardAxis=+Z  TranslationStandardOffset=0  TranslationStandardOffsetUnits=m  TranslationROffset=0  TranslationROffsetUnits=m  TranslationThetaOffset=0  TranslationThetaOffsetUnits=deg  TranslationZOffset=0  TranslationZOffsetUnits=m
  disque-1 (roue 1) : sm_lib/Body Elements/File Solid  Description=|  ExtGeomFileName=disque.stl  UnitType=Custom  ExtGeomFileUnits=mm  StepReaderType=HEX  ExportConvexHullGeometry=off  InertiaType=Custom  BasedOnType=DensityFromFile  Density=1000  DensityUnits=kg/m^3  Mass=0.027339457  MassUnits=kg  CenterOfMass=[3.5840173e-18 -4.1025221e-18 0.00225]  CenterOfMassUnits=m  MomentsOfInertia=[3.0147281e-05 3.0147281e-05 6.0202291e-05]  MomentsOfInertiaUnits=kg*m^2  ProductsOfInertia=[3.9369464e-23 -4.3624716e-23 -7.0860886e-22]  ProductsOfInertiaUnits=kg*m^2  GraphicType=FromGeometry  MarkerShape=Sphere  MarkerSize=10  GraphicVisPropType=SimpleVisualProperties  GraphicDiffuseColor=[0.769 0.306 0.322]  GraphicOpacity=1  GraphicSpecularColor=[0.5 0.5 0.5 1.0]  GraphicAmbientColor=[0.15 0.15 0.15 1.0]  GraphicEmissiveColor=[0.0 0.0 0.0 1.0]  GraphicShininess=75  DoExposeReferenceFrame=on  SerializedFrames=<Frames/>
      | Pièce CAO : disque-1 (roue 1) (disque)
      | Masse 27.34 g : PLA, plein × 0,9 (même hypothèse que le TP1), 1116 kg/m³.
      | Centre de masse et inertie : calculés sur la géométrie de la CAO.
  ecrous-1 (roue 1) : sm_lib/Body Elements/File Solid  Description=|  ExtGeomFileName=ecrous.stl  UnitType=Custom  ExtGeomFileUnits=mm  StepReaderType=HEX  ExportConvexHullGeometry=off  InertiaType=Custom  BasedOnType=DensityFromFile  Density=1000  DensityUnits=kg/m^3  Mass=0.0027655409  MassUnits=kg  CenterOfMass=[3.1829158e-19 0 0.003]  CenterOfMassUnits=m  MomentsOfInertia=[3.7203439e-08 3.7203439e-08 5.7813632e-08]  MomentsOfInertiaUnits=kg*m^2  ProductsOfInertia=[-1.9726372e-40 -8.2344948e-41 -7.5517615e-41]  ProductsOfInertiaUnits=kg*m^2  GraphicType=FromGeometry  MarkerShape=Sphere  MarkerSize=10  GraphicVisPropType=SimpleVisualProperties  GraphicDiffuseColor=[0.439 0.439 0.439]  GraphicOpacity=1  GraphicSpecularColor=[0.5 0.5 0.5 1.0]  GraphicAmbientColor=[0.15 0.15 0.15 1.0]  GraphicEmissiveColor=[0.0 0.0 0.0 1.0]  GraphicShininess=75  DoExposeReferenceFrame=on  SerializedFrames=<Frames/>
      | Pièce CAO : ecrous-1 (roue 1) (ecrous)
      | Masse 2.77 g : acier, 7850 kg/m³.
      | Centre de masse et inertie : calculés sur la géométrie de la CAO.
  ecrous-2 (roue 1) : sm_lib/Body Elements/File Solid  Description=|  ExtGeomFileName=ecrous.stl  UnitType=Custom  ExtGeomFileUnits=mm  StepReaderType=HEX  ExportConvexHullGeometry=off  InertiaType=Custom  BasedOnType=DensityFromFile  Density=1000  DensityUnits=kg/m^3  Mass=0.0027655409  MassUnits=kg  CenterOfMass=[3.1829158e-19 0 0.003]  CenterOfMassUnits=m  MomentsOfInertia=[3.7203439e-08 3.7203439e-08 5.7813632e-08]  MomentsOfInertiaUnits=kg*m^2  ProductsOfInertia=[-1.9726372e-40 -8.2344948e-41 -7.5517615e-41]  ProductsOfInertiaUnits=kg*m^2  GraphicType=FromGeometry  MarkerShape=Sphere  MarkerSize=10  GraphicVisPropType=SimpleVisualProperties  GraphicDiffuseColor=[0.439 0.439 0.439]  GraphicOpacity=1  GraphicSpecularColor=[0.5 0.5 0.5 1.0]  GraphicAmbientColor=[0.15 0.15 0.15 1.0]  GraphicEmissiveColor=[0.0 0.0 0.0 1.0]  GraphicShininess=75  DoExposeReferenceFrame=on  SerializedFrames=<Frames/>
      | Pièce CAO : ecrous-2 (roue 1) (ecrous)
      | Masse 2.77 g : acier, 7850 kg/m³.
      | Centre de masse et inertie : calculés sur la géométrie de la CAO.
  ecrous-3 (roue 1) : sm_lib/Body Elements/File Solid  Description=|  ExtGeomFileName=ecrous.stl  UnitType=Custom  ExtGeomFileUnits=mm  StepReaderType=HEX  ExportConvexHullGeometry=off  InertiaType=Custom  BasedOnType=DensityFromFile  Density=1000  DensityUnits=kg/m^3  Mass=0.0027655409  MassUnits=kg  CenterOfMass=[3.1829158e-19 0 0.003]  CenterOfMassUnits=m  MomentsOfInertia=[3.7203439e-08 3.7203439e-08 5.7813632e-08]  MomentsOfInertiaUnits=kg*m^2  ProductsOfInertia=[-1.9726372e-40 -8.2344948e-41 -7.5517615e-41]  ProductsOfInertiaUnits=kg*m^2  GraphicType=FromGeometry  MarkerShape=Sphere  MarkerSize=10  GraphicVisPropType=SimpleVisualProperties  GraphicDiffuseColor=[0.439 0.439 0.439]  GraphicOpacity=1  GraphicSpecularColor=[0.5 0.5 0.5 1.0]  GraphicAmbientColor=[0.15 0.15 0.15 1.0]  GraphicEmissiveColor=[0.0 0.0 0.0 1.0]  GraphicShininess=75  DoExposeReferenceFrame=on  SerializedFrames=<Frames/>
      | Pièce CAO : ecrous-3 (roue 1) (ecrous)
      | Masse 2.77 g : acier, 7850 kg/m³.
      | Centre de masse et inertie : calculés sur la géométrie de la CAO.
  ecrous-4 (roue 1) : sm_lib/Body Elements/File Solid  Description=|  ExtGeomFileName=ecrous.stl  UnitType=Custom  ExtGeomFileUnits=mm  StepReaderType=HEX  ExportConvexHullGeometry=off  InertiaType=Custom  BasedOnType=DensityFromFile  Density=1000  DensityUnits=kg/m^3  Mass=0.0027655409  MassUnits=kg  CenterOfMass=[3.1829158e-19 0 0.003]  CenterOfMassUnits=m  MomentsOfInertia=[3.7203439e-08 3.7203439e-08 5.7813632e-08]  MomentsOfInertiaUnits=kg*m^2  ProductsOfInertia=[-1.9726372e-40 -8.2344948e-41 -7.5517615e-41]  ProductsOfInertiaUnits=kg*m^2  GraphicType=FromGeometry  MarkerShape=Sphere  MarkerSize=10  GraphicVisPropType=SimpleVisualProperties  GraphicDiffuseColor=[0.439 0.439 0.439]  GraphicOpacity=1  GraphicSpecularColor=[0.5 0.5 0.5 1.0]  GraphicAmbientColor=[0.15 0.15 0.15 1.0]  GraphicEmissiveColor=[0.0 0.0 0.0 1.0]  GraphicShininess=75  DoExposeReferenceFrame=on  SerializedFrames=<Frames/>
      | Pièce CAO : ecrous-4 (roue 1) (ecrous)
      | Masse 2.77 g : acier, 7850 kg/m³.
      | Centre de masse et inertie : calculés sur la géométrie de la CAO.
  vis10-1 (roue 1) : sm_lib/Body Elements/File Solid  Description=|  ExtGeomFileName=vis10.stl  UnitType=Custom  ExtGeomFileUnits=mm  StepReaderType=HEX  ExportConvexHullGeometry=off  InertiaType=Custom  BasedOnType=DensityFromFile  Density=1000  DensityUnits=kg/m^3  Mass=0.003481639  MassUnits=kg  CenterOfMass=[4.3728344e-18 1.1656449e-19 0.0073902526]  CenterOfMassUnits=m  MomentsOfInertia=[6.4384479e-08 6.4384479e-08 1.9106608e-08]  MomentsOfInertiaUnits=kg*m^2  ProductsOfInertia=[-6.8499851e-25 -3.7892566e-23 -1.212724e-24]  ProductsOfInertiaUnits=kg*m^2  GraphicType=FromGeometry  MarkerShape=Sphere  MarkerSize=10  GraphicVisPropType=SimpleVisualProperties  GraphicDiffuseColor=[0.439 0.439 0.439]  GraphicOpacity=1  GraphicSpecularColor=[0.5 0.5 0.5 1.0]  GraphicAmbientColor=[0.15 0.15 0.15 1.0]  GraphicEmissiveColor=[0.0 0.0 0.0 1.0]  GraphicShininess=75  DoExposeReferenceFrame=on  SerializedFrames=<Frames/>
      | Pièce CAO : vis10-1 (roue 1) (vis10)
      | Masse 3.48 g : acier, 7850 kg/m³.
      | Centre de masse et inertie : calculés sur la géométrie de la CAO.
  vis10-2 (roue 1) : sm_lib/Body Elements/File Solid  Description=|  ExtGeomFileName=vis10.stl  UnitType=Custom  ExtGeomFileUnits=mm  StepReaderType=HEX  ExportConvexHullGeometry=off  InertiaType=Custom  BasedOnType=DensityFromFile  Density=1000  DensityUnits=kg/m^3  Mass=0.003481639  MassUnits=kg  CenterOfMass=[4.3728344e-18 1.1656449e-19 0.0073902526]  CenterOfMassUnits=m  MomentsOfInertia=[6.4384479e-08 6.4384479e-08 1.9106608e-08]  MomentsOfInertiaUnits=kg*m^2  ProductsOfInertia=[-6.8499851e-25 -3.7892566e-23 -1.212724e-24]  ProductsOfInertiaUnits=kg*m^2  GraphicType=FromGeometry  MarkerShape=Sphere  MarkerSize=10  GraphicVisPropType=SimpleVisualProperties  GraphicDiffuseColor=[0.439 0.439 0.439]  GraphicOpacity=1  GraphicSpecularColor=[0.5 0.5 0.5 1.0]  GraphicAmbientColor=[0.15 0.15 0.15 1.0]  GraphicEmissiveColor=[0.0 0.0 0.0 1.0]  GraphicShininess=75  DoExposeReferenceFrame=on  SerializedFrames=<Frames/>
      | Pièce CAO : vis10-2 (roue 1) (vis10)
      | Masse 3.48 g : acier, 7850 kg/m³.
      | Centre de masse et inertie : calculés sur la géométrie de la CAO.
  vis20-1 (roue 1) : sm_lib/Body Elements/File Solid  Description=|  ExtGeomFileName=vis20.stl  UnitType=Custom  ExtGeomFileUnits=mm  StepReaderType=HEX  ExportConvexHullGeometry=off  InertiaType=Custom  BasedOnType=DensityFromFile  Density=1000  DensityUnits=kg/m^3  Mass=0.0064718461  MassUnits=kg  CenterOfMass=[2.390239e-18 -6.2707839e-20 0.012260949]  CenterOfMassUnits=m  MomentsOfInertia=[3.2989031e-07 3.2989031e-07 3.6632652e-08]  MomentsOfInertiaUnits=kg*m^2  ProductsOfInertia=[3.1154167e-24 -1.1458442e-22 -6.862747e-24]  ProductsOfInertiaUnits=kg*m^2  GraphicType=FromGeometry  MarkerShape=Sphere  MarkerSize=10  GraphicVisPropType=SimpleVisualProperties  GraphicDiffuseColor=[0.439 0.439 0.439]  GraphicOpacity=1  GraphicSpecularColor=[0.5 0.5 0.5 1.0]  GraphicAmbientColor=[0.15 0.15 0.15 1.0]  GraphicEmissiveColor=[0.0 0.0 0.0 1.0]  GraphicShininess=75  DoExposeReferenceFrame=on  SerializedFrames=<Frames/>
      | Pièce CAO : vis20-1 (roue 1) (vis20)
      | Masse 6.47 g : acier, 7850 kg/m³.
      | Centre de masse et inertie : calculés sur la géométrie de la CAO.
  vis20-2 (roue 1) : sm_lib/Body Elements/File Solid  Description=|  ExtGeomFileName=vis20.stl  UnitType=Custom  ExtGeomFileUnits=mm  StepReaderType=HEX  ExportConvexHullGeometry=off  InertiaType=Custom  BasedOnType=DensityFromFile  Density=1000  DensityUnits=kg/m^3  Mass=0.0064718461  MassUnits=kg  CenterOfMass=[2.390239e-18 -6.2707839e-20 0.012260949]  CenterOfMassUnits=m  MomentsOfInertia=[3.2989031e-07 3.2989031e-07 3.6632652e-08]  MomentsOfInertiaUnits=kg*m^2  ProductsOfInertia=[3.1154167e-24 -1.1458442e-22 -6.862747e-24]  ProductsOfInertiaUnits=kg*m^2  GraphicType=FromGeometry  MarkerShape=Sphere  MarkerSize=10  GraphicVisPropType=SimpleVisualProperties  GraphicDiffuseColor=[0.439 0.439 0.439]  GraphicOpacity=1  GraphicSpecularColor=[0.5 0.5 0.5 1.0]  GraphicAmbientColor=[0.15 0.15 0.15 1.0]  GraphicEmissiveColor=[0.0 0.0 0.0 1.0]  GraphicShininess=75  DoExposeReferenceFrame=on  SerializedFrames=<Frames/>
      | Pièce CAO : vis20-2 (roue 1) (vis20)
      | Masse 6.47 g : acier, 7850 kg/m³.
      | Centre de masse et inertie : calculés sur la géométrie de la CAO.
  F : PMIOPort  Side=Left
  connections:
  Pose A2212 rotor (roue 1)/LConn1 -- F/RConn1 -- Pose ecrous-2 (roue 1)/LConn1 -- Pose vis10-1 (roue 1)/LConn1 -- Pose vis10-2 (roue 1)/LConn1 -- Pose ecrous-1 (roue 1)/LConn1 -- Pose vis20-1 (roue 1)/LConn1 -- Pose vis20-2 (roue 1)/LConn1 -- Pose ecrous-3 (roue 1)/LConn1 -- Pose disque-1 (roue 1)/LConn1 -- Pose ecrous-4 (roue 1)/LConn1
  Pose A2212 rotor (roue 1)/RConn1 -- A2212 rotor (roue 1)/RConn1
  Pose ecrous-2 (roue 1)/RConn1 -- ecrous-2 (roue 1)/RConn1
  Pose vis10-1 (roue 1)/RConn1 -- vis10-1 (roue 1)/RConn1
  Pose vis10-2 (roue 1)/RConn1 -- vis10-2 (roue 1)/RConn1
  Pose ecrous-1 (roue 1)/RConn1 -- ecrous-1 (roue 1)/RConn1
  Pose vis20-1 (roue 1)/RConn1 -- vis20-1 (roue 1)/RConn1
  Pose vis20-2 (roue 1)/RConn1 -- vis20-2 (roue 1)/RConn1
  Pose ecrous-3 (roue 1)/RConn1 -- ecrous-3 (roue 1)/RConn1
  Pose disque-1 (roue 1)/RConn1 -- disque-1 (roue 1)/RConn1
  Pose ecrous-4 (roue 1)/RConn1 -- ecrous-4 (roue 1)/RConn1
